simulink model "microgrid_4dg"  (R2025a)
settings: Solver=FixedStepDiscrete  StartTime=0.0  StopTime=0.4  FixedStep=2.5e-06  RelTol=1e-3
libraries: spsThreePhaseSeriesRLCBranchLib x16, spsNeutralLib x10, spsThreePhaseBreakerLib x9, spsThreePhaseVIMeasurementLib x8, spsPWMGenerator2LevelLib x4, spsDCVoltageSourceLib x4, spsUniversalBridgeLib x4, spsGroundLib x1, spspowerguiLib x1
settings Model: Creator=mahmudakon  LastModifiedBy=mahmudakon

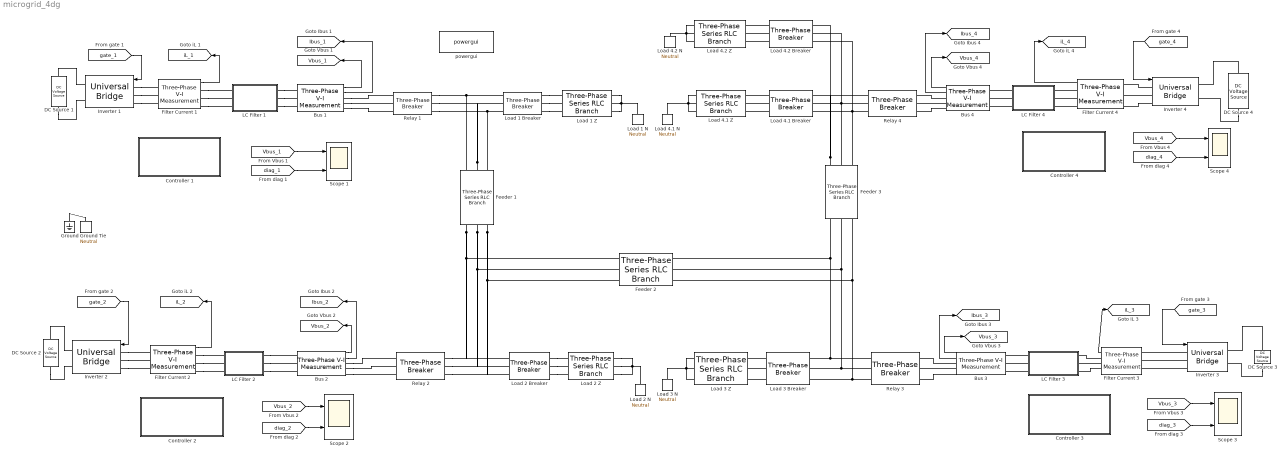
== system microgrid_4dg ==
  Bus {1..4} (4 alike) : spsThreePhaseVIMeasurementLib/Three-Phase V-I Measurement  VoltageMeasurement=phase-to-ground  SetLabelV=off  LabelV=Vabc  Vpu=off  VpuLL=off  CurrentMeasurement=yes  SetLabelI=off  LabelI=Iabc  Ipu=off  Pbase=100e6  Vbase=500e3  OutputType=Complex  PhasorSimulation=off  PSBequivalent=0
  Controller 1 : Subsystem
  Controller 2 : Subsystem
  Controller 3 : Subsystem
  Controller 4 : Subsystem
  DC Source {1..4} (4 alike) : spsDCVoltageSourceLib/DC Voltage Source  Amplitude=45  Measurements=None
  Feeder 1 : spsThreePhaseSeriesRLCBranchLib/Three-Phase Series RLC Branch  LConnTagsString=A|B|C  RConnTagsString=A|B|C  BranchType=RL  Resistance=0.13  Inductance=3.3e-6  Capacitance=1e-6  Measurements=None
  Feeder 2 : spsThreePhaseSeriesRLCBranchLib/Three-Phase Series RLC Branch  LConnTagsString=A|B|C  RConnTagsString=A|B|C  BranchType=RL  Resistance=0.13  Inductance=3.3e-6  Capacitance=1e-6  Measurements=None
  Feeder 3 : spsThreePhaseSeriesRLCBranchLib/Three-Phase Series RLC Branch  LConnTagsString=A|B|C  RConnTagsString=A|B|C  BranchType=RL  Resistance=0.13  Inductance=3.3e-6  Capacitance=1e-6  Measurements=None
  Filter Current {1..4} (4 alike) : spsThreePhaseVIMeasurementLib/Three-Phase V-I Measurement  VoltageMeasurement=no  SetLabelV=off  LabelV=Vabc  Vpu=off  VpuLL=off  CurrentMeasurement=yes  SetLabelI=off  LabelI=Iabc  Ipu=off  Pbase=100e6  Vbase=500e3  OutputType=Complex  PhasorSimulation=off  PSBequivalent=0
  Ground : spsGroundLib/Ground  LConnTagsString=a
  Ground Tie : spsNeutralLib/Neutral  LConnTagsString=a  NodeNumber=1
      settings: AttributesFormatString=node %<NodeNumber>  LibrarySourceBlock=sps_lib/Utilities/Neutral
  Inverter {1..4} (4 alike) : spsUniversalBridgeLib/Universal Bridge  Arms=3  SnubberResistance=1e5  SnubberCapacitance=inf  Device=IGBT / Diodes  Ron=1e-3  Lon=0  ForwardVoltages="[  0  0  ]"  ForwardVoltage=0  GTOparameters=[ 10e-6 , 20e-6 ]  IGBTparameters=[ 1e-6 , 2e-6 ]  Measurements=None  Measurements_2=None  converterType=Rectifier
  LC Filter 1 : Subsystem
  LC Filter 2 : Subsystem
  LC Filter 3 : Subsystem
  LC Filter 4 : Subsystem
  Load 1 Breaker : spsThreePhaseBreakerLib/Three-Phase Breaker  InitialState=closed  SwitchA=on  SwitchB=on  SwitchC=on  SwitchTimes=[1e6]  External=off  BreakerResistance=0.01  SnubberResistance=1e6  SnubberCapacitance=inf  Measurements=None
  Load 1 N : spsNeutralLib/Neutral  LConnTagsString=a  NodeNumber=1
      settings: AttributesFormatString=node %<NodeNumber>  LibrarySourceBlock=sps_lib/Utilities/Neutral
  Load 1 Z : spsThreePhaseSeriesRLCBranchLib/Three-Phase Series RLC Branch  LConnTagsString=A|B|C  RConnTagsString=A|B|C  BranchType=RL  Resistance=10.08  Inductance=6.25e-3  Capacitance=1e-6  Measurements=None
  Load 2 Breaker : spsThreePhaseBreakerLib/Three-Phase Breaker  InitialState=closed  SwitchA=on  SwitchB=on  SwitchC=on  SwitchTimes=[1e6]  External=off  BreakerResistance=0.01  SnubberResistance=1e6  SnubberCapacitance=inf  Measurements=None
  Load 2 N : spsNeutralLib/Neutral  LConnTagsString=a  NodeNumber=2
      settings: AttributesFormatString=node %<NodeNumber>  LibrarySourceBlock=sps_lib/Utilities/Neutral
  Load 2 Z : spsThreePhaseSeriesRLCBranchLib/Three-Phase Series RLC Branch  LConnTagsString=A|B|C  RConnTagsString=A|B|C  BranchType=RL  Resistance=28.34  Inductance=8.00e-3  Capacitance=1e-6  Measurements=None
  Load 3 Breaker : spsThreePhaseBreakerLib/Three-Phase Breaker  InitialState=closed  SwitchA=on  SwitchB=on  SwitchC=on  SwitchTimes=[1e6]  External=off  BreakerResistance=0.01  SnubberResistance=1e6  SnubberCapacitance=inf  Measurements=None
  Load 3 N : spsNeutralLib/Neutral  LConnTagsString=a  NodeNumber=3
      settings: AttributesFormatString=node %<NodeNumber>  LibrarySourceBlock=sps_lib/Utilities/Neutral
  Load 3 Z : spsThreePhaseSeriesRLCBranchLib/Three-Phase Series RLC Branch  LConnTagsString=A|B|C  RConnTagsString=A|B|C  BranchType=RL  Resistance=25.56  Inductance=1.80e-3  Capacitance=1e-6  Measurements=None
  Load 4.1 Breaker : spsThreePhaseBreakerLib/Three-Phase Breaker  InitialState=closed  SwitchA=on  SwitchB=on  SwitchC=on  SwitchTimes=[1e6]  External=off  BreakerResistance=0.01  SnubberResistance=1e6  SnubberCapacitance=inf  Measurements=None
  Load 4.1 N : spsNeutralLib/Neutral  LConnTagsString=a  NodeNumber=4
      settings: AttributesFormatString=node %<NodeNumber>  LibrarySourceBlock=sps_lib/Utilities/Neutral
  Load 4.1 Z : spsThreePhaseSeriesRLCBranchLib/Three-Phase Series RLC Branch  LConnTagsString=A|B|C  RConnTagsString=A|B|C  BranchType=RL  Resistance=10.08  Inductance=6.25e-3  Capacitance=1e-6  Measurements=None
  Load 4.2 Breaker : spsThreePhaseBreakerLib/Three-Phase Breaker  InitialState=open  SwitchA=on  SwitchB=on  SwitchC=on  SwitchTimes=0.2  External=off  BreakerResistance=0.01  SnubberResistance=1e6  SnubberCapacitance=inf  Measurements=None
  Load 4.2 N : spsNeutralLib/Neutral  LConnTagsString=a  NodeNumber=4
      settings: AttributesFormatString=node %<NodeNumber>  LibrarySourceBlock=sps_lib/Utilities/Neutral
  Load 4.2 Z : spsThreePhaseSeriesRLCBranchLib/Three-Phase Series RLC Branch  LConnTagsString=A|B|C  RConnTagsString=A|B|C  BranchType=R  Resistance=10  Inductance=1e-3  Capacitance=1e-6  Measurements=None
  Relay {1..4} (4 alike) : spsThreePhaseBreakerLib/Three-Phase Breaker  InitialState=closed  SwitchA=on  SwitchB=on  SwitchC=on  SwitchTimes=[1e6]  External=off  BreakerResistance=0.01  SnubberResistance=1e6  SnubberCapacitance=inf  Measurements=None
  Scope {1..4} (4 alike) : Scope  NumInputPorts=2
      Scope 1 settings: ActiveDisplayYMinimum=12.426421052352524  ActiveDisplayYMaximum=163.05760904851627
      Scope 4 settings: ActiveDisplayYMinimum=-55.5325630889955  ActiveDisplayYMaximum=59.486517619510956
  powergui : spspowerguiLib/powergui  Priority=1  SimulationMode=Discrete  SampleTime=2.5e-06  frequency=60  Iterations=50  frequencyindice=0  Pbase=100e6  ErrMax=1e-4  UnitsV=kV  UnitsW=MW  buscounter=0  FunctionMessages=off  echomessages=off  EnableUseOfTLC=off  CurrentSourceSwitches=off  DisableSnubberDevices=off  DisableRonSwitches=off  DisableVfSwitches=off  DisplayEquations=off  AutomaticDiscreteSolvers=off  SolverType=Tustin/Backward Euler (TBE)  Interpol=off  ExternalGateDelay=off  methode=off  Ts=100  x0status=blocks  SPID=on  SwTol=0  HookPort=off  NonlinearTolerance=1e-4  nMaxIteration=100  ContinueOnMaxIteration=off  RestoreLinks=warning  ResistiveCurrentMeasurement=off  Frange=[0:2:500]  Ylog=off  Xlog=on  ShowGrid=off  save=off  variable=ZData  structure=0  ZoomFFT=off  StartTime=0.0  cycles=1  DisplayStyle=1  fundamental=60  FreqAxis=off  MaxFrequency=1000  frequencyindicesteady=1  RmsSteady=1  display=off
  tag scope: Ibus_1=global, Ibus_2=global, Ibus_3=global, Ibus_4=global, Vbus_1=global, Vbus_2=global, Vbus_3=global, Vbus_4=global, iL_1=global, iL_2=global, iL_3=global, iL_4=global
  wires:
  Filter Current 1/1 -> [iL_1]
  Bus 1/1 -> [Vbus_1]
  Bus 1/2 -> [Ibus_1]
  [gate_1] -> Inverter 1/1
  Filter Current 2/1 -> [iL_2]
  Bus 2/1 -> [Vbus_2]
  Bus 2/2 -> [Ibus_2]
  [gate_2] -> Inverter 2/1
  Filter Current 3/1 -> [iL_3]
  Bus 3/1 -> [Vbus_3]
  Bus 3/2 -> [Ibus_3]
  [gate_3] -> Inverter 3/1
  Filter Current 4/1 -> [iL_4]
  Bus 4/1 -> [Vbus_4]
  Bus 4/2 -> [Ibus_4]
  [gate_4] -> Inverter 4/1
  [Vbus_1] -> Scope 1/1
  [diag_1] -> Scope 1/2
  [Vbus_2] -> Scope 2/1
  [diag_2] -> Scope 2/2
  [Vbus_3] -> Scope 3/1
  [diag_3] -> Scope 3/2
  [Vbus_4] -> Scope 4/1
  [diag_4] -> Scope 4/2
  connections:
  Ground/LConn1 -- Ground Tie/LConn1
  DC Source 1/RConn1 -- Inverter 1/RConn1
  DC Source 1/LConn1 -- Inverter 1/RConn2
  Inverter 1/LConn1 -- Filter Current 1/LConn1
  Filter Current 1/RConn1 -- LC Filter 1/LConn1
  LC Filter 1/RConn1 -- Bus 1/LConn1
  Bus 1/RConn1 -- Relay 1/LConn1
  Inverter 1/LConn2 -- Filter Current 1/LConn2
  Filter Current 1/RConn2 -- LC Filter 1/LConn2
  LC Filter 1/RConn2 -- Bus 1/LConn2
  Bus 1/RConn2 -- Relay 1/LConn2
  Inverter 1/LConn3 -- Filter Current 1/LConn3
  Filter Current 1/RConn3 -- LC Filter 1/LConn3
  LC Filter 1/RConn3 -- Bus 1/LConn3
  Bus 1/RConn3 -- Relay 1/LConn3
  DC Source 2/RConn1 -- Inverter 2/RConn1
  DC Source 2/LConn1 -- Inverter 2/RConn2
  Inverter 2/LConn1 -- Filter Current 2/LConn1
  Filter Current 2/RConn1 -- LC Filter 2/LConn1
  LC Filter 2/RConn1 -- Bus 2/LConn1
  Bus 2/RConn1 -- Relay 2/LConn1
  Inverter 2/LConn2 -- Filter Current 2/LConn2
  Filter Current 2/RConn2 -- LC Filter 2/LConn2
  LC Filter 2/RConn2 -- Bus 2/LConn2
  Bus 2/RConn2 -- Relay 2/LConn2
  Inverter 2/LConn3 -- Filter Current 2/LConn3
  Filter Current 2/RConn3 -- LC Filter 2/LConn3
  LC Filter 2/RConn3 -- Bus 2/LConn3
  Bus 2/RConn3 -- Relay 2/LConn3
  DC Source 3/RConn1 -- Inverter 3/RConn1
  DC Source 3/LConn1 -- Inverter 3/RConn2
  Inverter 3/LConn1 -- Filter Current 3/LConn1
  Filter Current 3/RConn1 -- LC Filter 3/LConn1
  LC Filter 3/RConn1 -- Bus 3/LConn1
  Bus 3/RConn1 -- Relay 3/LConn1
  Inverter 3/LConn2 -- Filter Current 3/LConn2
  Filter Current 3/RConn2 -- LC Filter 3/LConn2
  LC Filter 3/RConn2 -- Bus 3/LConn2
  Bus 3/RConn2 -- Relay 3/LConn2
  Inverter 3/LConn3 -- Filter Current 3/LConn3
  Filter Current 3/RConn3 -- LC Filter 3/LConn3
  LC Filter 3/RConn3 -- Bus 3/LConn3
  Bus 3/RConn3 -- Relay 3/LConn3
  DC Source 4/RConn1 -- Inverter 4/RConn1
  DC Source 4/LConn1 -- Inverter 4/RConn2
  Inverter 4/LConn1 -- Filter Current 4/LConn1
  Filter Current 4/RConn1 -- LC Filter 4/LConn1
  LC Filter 4/RConn1 -- Bus 4/LConn1
  Bus 4/RConn1 -- Relay 4/LConn1
  Inverter 4/LConn2 -- Filter Current 4/LConn2
  Filter Current 4/RConn2 -- LC Filter 4/LConn2
  LC Filter 4/RConn2 -- Bus 4/LConn2
  Bus 4/RConn2 -- Relay 4/LConn2
  Inverter 4/LConn3 -- Filter Current 4/LConn3
  Filter Current 4/RConn3 -- LC Filter 4/LConn3
  LC Filter 4/RConn3 -- Bus 4/LConn3
  Bus 4/RConn3 -- Relay 4/LConn3
  Relay 1/RConn1 -- Load 1 Breaker/LConn1 -- Feeder 1/LConn1
  Feeder 1/RConn1 -- Load 2 Breaker/LConn1 -- Relay 2/RConn1 -- Feeder 2/LConn1
  Feeder 1/LConn2 -- Relay 1/RConn2 -- Load 1 Breaker/LConn2
  Feeder 1/RConn2 -- Load 2 Breaker/LConn2 -- Relay 2/RConn2 -- Feeder 2/LConn2
  Relay 1/RConn3 -- Feeder 1/LConn3 -- Load 1 Breaker/LConn3
  Feeder 1/RConn3 -- Load 2 Breaker/LConn3 -- Relay 2/RConn3 -- Feeder 2/LConn3
  Relay 3/RConn1 -- Feeder 3/LConn1 -- Feeder 2/RConn1 -- Load 3 Breaker/LConn1
  Relay 3/RConn2 -- Feeder 3/LConn2 -- Feeder 2/RConn2 -- Load 3 Breaker/LConn2
  Relay 3/RConn3 -- Feeder 3/LConn3 -- Feeder 2/RConn3 -- Load 3 Breaker/LConn3
  Feeder 3/RConn1 -- Load 4.2 Breaker/LConn1 -- Relay 4/RConn1 -- Load 4.1 Breaker/LConn1
  Relay 4/RConn2 -- Load 4.2 Breaker/LConn2 -- Feeder 3/RConn2 -- Load 4.1 Breaker/LConn2
  Relay 4/RConn3 -- Load 4.2 Breaker/LConn3 -- Load 4.1 Breaker/LConn3 -- Feeder 3/RConn3
  Load 1 Breaker/RConn1 -- Load 1 Z/LConn1
  Load 1 Z/RConn1 -- Load 1 Z/RConn3 -- Load 1 Z/RConn2 -- Load 1 N/LConn1
  Load 1 Breaker/RConn2 -- Load 1 Z/LConn2
  Load 1 Breaker/RConn3 -- Load 1 Z/LConn3
  Load 2 Breaker/RConn1 -- Load 2 Z/LConn1
  Load 2 Z/RConn1 -- Load 2 Z/RConn3 -- Load 2 N/LConn1 -- Load 2 Z/RConn2
  Load 2 Breaker/RConn2 -- Load 2 Z/LConn2
  Load 2 Breaker/RConn3 -- Load 2 Z/LConn3
  Load 3 Breaker/RConn1 -- Load 3 Z/LConn1
  Load 3 Z/RConn1 -- Load 3 N/LConn1 -- Load 3 Z/RConn3 -- Load 3 Z/RConn2
  Load 3 Breaker/RConn2 -- Load 3 Z/LConn2
  Load 3 Breaker/RConn3 -- Load 3 Z/LConn3
  Load 4.1 Breaker/RConn1 -- Load 4.1 Z/LConn1
  Load 4.1 Z/RConn1 -- Load 4.1 N/LConn1 -- Load 4.1 Z/RConn3 -- Load 4.1 Z/RConn2
  Load 4.1 Breaker/RConn2 -- Load 4.1 Z/LConn2
  Load 4.1 Breaker/RConn3 -- Load 4.1 Z/LConn3
  Load 4.2 Breaker/RConn1 -- Load 4.2 Z/LConn1
  Load 4.2 Z/RConn1 -- Load 4.2 Z/RConn3 -- Load 4.2 N/LConn1 -- Load 4.2 Z/RConn2
  Load 4.2 Breaker/RConn2 -- Load 4.2 Z/LConn2
  Load 4.2 Breaker/RConn3 -- Load 4.2 Z/LConn3

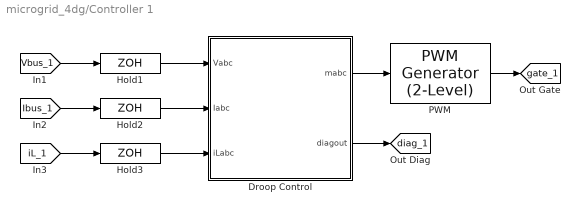
== system microgrid_4dg/Controller 1 ==
  Droop Control : MATLAB Function  TreatAsAtomicUnit=on
  Hold1 : ZeroOrderHold  SampleTime=50e-6
  Hold2 : ZeroOrderHold  SampleTime=50e-6
  Hold3 : ZeroOrderHold  SampleTime=50e-6
  PWM : spsPWMGenerator2LevelLib/PWM Generator (2-Level)  ModulatorType=Three-phase bridge (6 pulses)  ModulatorMode=Unsynchronized  Fc=20000  Pc=90  nF=27  MinMax="[ -1  1 ]"  SamplingTechnique=Natural  ModulatingSignals=off  m=0.8  Freq=60  Phase=0  Ts=0  ShowCarrierOutport=off
  tag scope: diag_1=global, gate_1=global
  wires:
  Hold3/1 -> Droop Control/3(iLabc)
  Droop Control/1(mabc) -> PWM/1
  [iL_1] -> Hold3/1
  Hold1/1 -> Droop Control/1(Vabc)
  [Ibus_1] -> Hold2/1
  Droop Control/2(diagout) -> [diag_1]
  Hold2/1 -> Droop Control/2(Iabc)
  PWM/1 -> [gate_1]
  [Vbus_1] -> Hold1/1

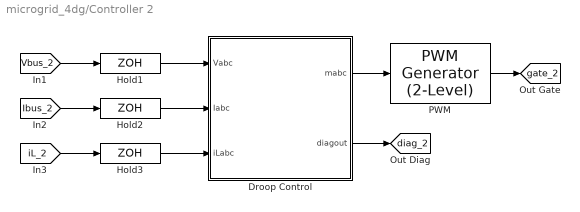
== system microgrid_4dg/Controller 2 ==
  Droop Control : MATLAB Function  TreatAsAtomicUnit=on
  Hold1 : ZeroOrderHold  SampleTime=50e-6
  Hold2 : ZeroOrderHold  SampleTime=50e-6
  Hold3 : ZeroOrderHold  SampleTime=50e-6
  PWM : spsPWMGenerator2LevelLib/PWM Generator (2-Level)  ModulatorType=Three-phase bridge (6 pulses)  ModulatorMode=Unsynchronized  Fc=20000  Pc=90  nF=27  MinMax="[ -1  1 ]"  SamplingTechnique=Natural  ModulatingSignals=off  m=0.8  Freq=60  Phase=0  Ts=0  ShowCarrierOutport=off
  tag scope: diag_2=global, gate_2=global
  wires:
  Hold3/1 -> Droop Control/3(iLabc)
  Droop Control/2(diagout) -> [diag_2]
  [iL_2] -> Hold3/1
  Droop Control/1(mabc) -> PWM/1
  Hold1/1 -> Droop Control/1(Vabc)
  [Ibus_2] -> Hold2/1
  Hold2/1 -> Droop Control/2(Iabc)
  PWM/1 -> [gate_2]
  [Vbus_2] -> Hold1/1

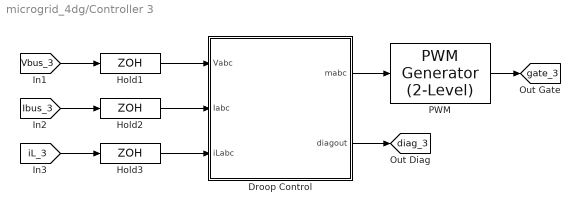
== system microgrid_4dg/Controller 3 ==
  Droop Control : MATLAB Function  TreatAsAtomicUnit=on
  Hold1 : ZeroOrderHold  SampleTime=50e-6
  Hold2 : ZeroOrderHold  SampleTime=50e-6
  Hold3 : ZeroOrderHold  SampleTime=50e-6
  PWM : spsPWMGenerator2LevelLib/PWM Generator (2-Level)  ModulatorType=Three-phase bridge (6 pulses)  ModulatorMode=Unsynchronized  Fc=20000  Pc=90  nF=27  MinMax="[ -1  1 ]"  SamplingTechnique=Natural  ModulatingSignals=off  m=0.8  Freq=60  Phase=0  Ts=0  ShowCarrierOutport=off
  tag scope: diag_3=global, gate_3=global
  wires:
  Hold3/1 -> Droop Control/3(iLabc)
  Droop Control/2(diagout) -> [diag_3]
  [iL_3] -> Hold3/1
  Droop Control/1(mabc) -> PWM/1
  Hold1/1 -> Droop Control/1(Vabc)
  [Ibus_3] -> Hold2/1
  Hold2/1 -> Droop Control/2(Iabc)
  PWM/1 -> [gate_3]
  [Vbus_3] -> Hold1/1

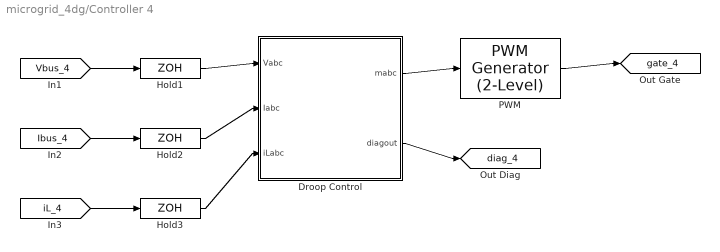
== system microgrid_4dg/Controller 4 ==
  Droop Control : MATLAB Function  TreatAsAtomicUnit=on
  Hold1 : ZeroOrderHold  SampleTime=50e-6
  Hold2 : ZeroOrderHold  SampleTime=50e-6
  Hold3 : ZeroOrderHold  SampleTime=50e-6
  PWM : spsPWMGenerator2LevelLib/PWM Generator (2-Level)  ModulatorType=Three-phase bridge (6 pulses)  ModulatorMode=Unsynchronized  Fc=20000  Pc=90  nF=27  MinMax="[ -1  1 ]"  SamplingTechnique=Natural  ModulatingSignals=off  m=0.8  Freq=60  Phase=0  Ts=0  ShowCarrierOutport=off
  tag scope: diag_4=global, gate_4=global
  wires:
  [Vbus_4] -> Hold1/1
  [Ibus_4] -> Hold2/1
  [iL_4] -> Hold3/1
  Hold1/1 -> Droop Control/1(Vabc)
  Hold2/1 -> Droop Control/2(Iabc)
  Hold3/1 -> Droop Control/3(iLabc)
  Droop Control/1(mabc) -> PWM/1
  PWM/1 -> [gate_4]
  Droop Control/2(diagout) -> [diag_4]

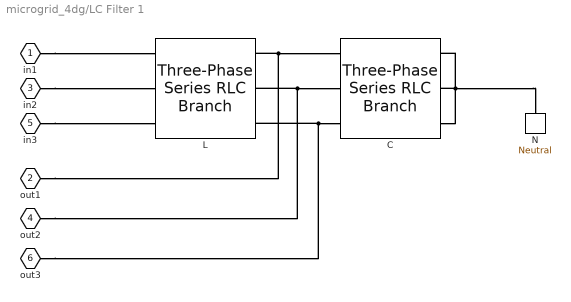
== system microgrid_4dg/LC Filter 1 ==
  C : spsThreePhaseSeriesRLCBranchLib/Three-Phase Series RLC Branch  LConnTagsString=A|B|C  RConnTagsString=A|B|C  BranchType=C  Resistance=1  Inductance=1e-3  Capacitance=22e-6  Measurements=None
  L : spsThreePhaseSeriesRLCBranchLib/Three-Phase Series RLC Branch  LConnTagsString=A|B|C  RConnTagsString=A|B|C  BranchType=L  Resistance=1  Inductance=0.56e-3  Capacitance=1e-6  Measurements=None
  N : spsNeutralLib/Neutral  LConnTagsString=a  NodeNumber=1
      settings: AttributesFormatString=node %<NodeNumber>  LibrarySourceBlock=sps_lib/Utilities/Neutral
  in1 : PMIOPort  Side=Left
  out1 : PMIOPort  Port=2  Side=Right
  in2 : PMIOPort  Port=3  Side=Left
  out2 : PMIOPort  Port=4  Side=Right
  in3 : PMIOPort  Port=5  Side=Left
  out3 : PMIOPort  Port=6  Side=Right
  connections:
  out2/RConn1 -- C/LConn2 -- L/RConn2
  out1/RConn1 -- C/LConn1 -- L/RConn1
  in3/RConn1 -- L/LConn3
  in2/RConn1 -- L/LConn2
  out3/RConn1 -- L/RConn3 -- C/LConn3
  C/RConn3 -- N/LConn1 -- C/RConn1 -- C/RConn2
  in1/RConn1 -- L/LConn1

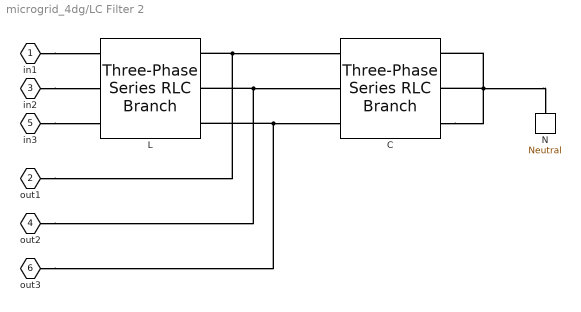
== system microgrid_4dg/LC Filter 2 ==
  C : spsThreePhaseSeriesRLCBranchLib/Three-Phase Series RLC Branch  LConnTagsString=A|B|C  RConnTagsString=A|B|C  BranchType=C  Resistance=1  Inductance=1e-3  Capacitance=22e-6  Measurements=None
  L : spsThreePhaseSeriesRLCBranchLib/Three-Phase Series RLC Branch  LConnTagsString=A|B|C  RConnTagsString=A|B|C  BranchType=L  Resistance=1  Inductance=0.56e-3  Capacitance=1e-6  Measurements=None
  N : spsNeutralLib/Neutral  LConnTagsString=a  NodeNumber=2
      settings: AttributesFormatString=node %<NodeNumber>  LibrarySourceBlock=sps_lib/Utilities/Neutral
  in1 : PMIOPort  Side=Left
  out1 : PMIOPort  Port=2  Side=Right
  in2 : PMIOPort  Port=3  Side=Left
  out2 : PMIOPort  Port=4  Side=Right
  in3 : PMIOPort  Port=5  Side=Left
  out3 : PMIOPort  Port=6  Side=Right
  connections:
  out3/RConn1 -- C/LConn3 -- L/RConn3
  out2/RConn1 -- C/LConn2 -- L/RConn2
  out1/RConn1 -- L/RConn1 -- C/LConn1
  in3/RConn1 -- L/LConn3
  in2/RConn1 -- L/LConn2
  C/RConn3 -- N/LConn1 -- C/RConn1 -- C/RConn2
  in1/RConn1 -- L/LConn1

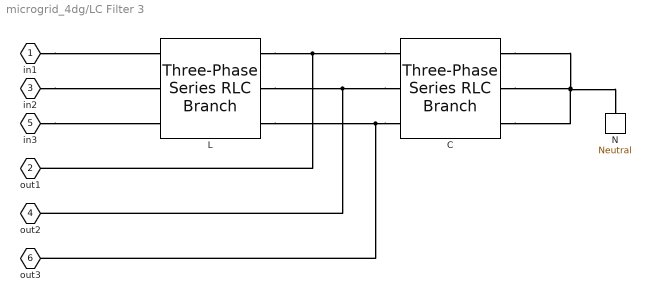
== system microgrid_4dg/LC Filter 3 ==
  C : spsThreePhaseSeriesRLCBranchLib/Three-Phase Series RLC Branch  LConnTagsString=A|B|C  RConnTagsString=A|B|C  BranchType=C  Resistance=1  Inductance=1e-3  Capacitance=22e-6  Measurements=None
  L : spsThreePhaseSeriesRLCBranchLib/Three-Phase Series RLC Branch  LConnTagsString=A|B|C  RConnTagsString=A|B|C  BranchType=L  Resistance=1  Inductance=0.56e-3  Capacitance=1e-6  Measurements=None
  N : spsNeutralLib/Neutral  LConnTagsString=a  NodeNumber=3
      settings: AttributesFormatString=node %<NodeNumber>  LibrarySourceBlock=sps_lib/Utilities/Neutral
  in1 : PMIOPort  Side=Left
  out1 : PMIOPort  Port=2  Side=Right
  in2 : PMIOPort  Port=3  Side=Left
  out2 : PMIOPort  Port=4  Side=Right
  in3 : PMIOPort  Port=5  Side=Left
  out3 : PMIOPort  Port=6  Side=Right
  connections:
  in1/RConn1 -- L/LConn1
  C/LConn1 -- L/RConn1 -- out1/RConn1
  C/RConn1 -- C/RConn3 -- N/LConn1 -- C/RConn2
  in2/RConn1 -- L/LConn2
  C/LConn2 -- L/RConn2 -- out2/RConn1
  in3/RConn1 -- L/LConn3
  C/LConn3 -- L/RConn3 -- out3/RConn1

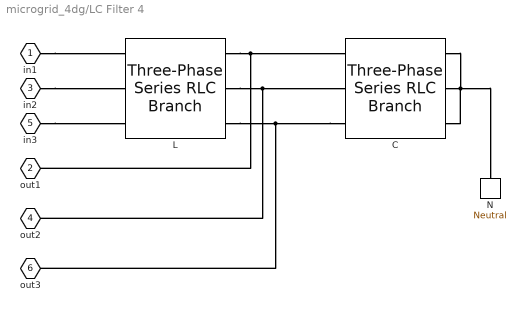
== system microgrid_4dg/LC Filter 4 ==
  C : spsThreePhaseSeriesRLCBranchLib/Three-Phase Series RLC Branch  LConnTagsString=A|B|C  RConnTagsString=A|B|C  BranchType=C  Resistance=1  Inductance=1e-3  Capacitance=22e-6  Measurements=None
  L : spsThreePhaseSeriesRLCBranchLib/Three-Phase Series RLC Branch  LConnTagsString=A|B|C  RConnTagsString=A|B|C  BranchType=L  Resistance=1  Inductance=0.56e-3  Capacitance=1e-6  Measurements=None
  N : spsNeutralLib/Neutral  LConnTagsString=a  NodeNumber=4
      settings: AttributesFormatString=node %<NodeNumber>  LibrarySourceBlock=sps_lib/Utilities/Neutral
  in1 : PMIOPort  Side=Left
  out1 : PMIOPort  Port=2  Side=Right
  in2 : PMIOPort  Port=3  Side=Left
  out2 : PMIOPort  Port=4  Side=Right
  in3 : PMIOPort  Port=5  Side=Left
  out3 : PMIOPort  Port=6  Side=Right
  connections:
  in1/RConn1 -- L/LConn1
  L/RConn1 -- C/LConn1 -- out1/RConn1
  C/RConn1 -- N/LConn1 -- C/RConn3 -- C/RConn2
  in2/RConn1 -- L/LConn2
  L/RConn2 -- C/LConn2 -- out2/RConn1
  in3/RConn1 -- L/LConn3
  C/LConn3 -- out3/RConn1 -- L/RConn3

== matlab function microgrid_4dg/Controller 2/Droop Control ==
  data: Vabc input; mabc output; Iabc input; iLabc input; diagout output
function [mabc, diagout] = dgctrl(Vabc, Iabc, iLabc)
persistent theta Pf Qf intVd intVq intId intIq inited
if isempty(inited)
    theta = 0; Pf = 0; Qf = 0;
    intVd = 0; intVq = 0; intId = 0; intIq = 0;
    inited = true;
end
dt = 5e-05;
w0 = 2*pi*60;
Vdc = 45;
Vnom = 18;
Lf = 0.00056;
Cf = 2.2e-05;
mp = 0.009424777961;
nq = 0.006;
wc = 2*pi*1;
kpv = 0.5; kiv = 200;
kpi = 15;  kii = 4000;
Lv = 0.003;   % virtual series inductance (Pogaku-style virtual impedance)
Kad = 0.5;  % active-damping gain on capacitor current (LC resonance damping)

[Vd, Vq]   = abc2dq(Vabc, theta);
[Id, Iq]   = abc2dq(Iabc, theta);
[ILd, ILq] = abc2dq(iLabc, theta);

Pinst = 1.5*(Vd*Id + Vq*Iq);
Qinst = 1.5*(Vq*Id - Vd*Iq);
Pf = Pf + dt*wc*(Pinst - Pf);
Qf = Qf + dt*wc*(Qinst - Qf);

w = w0 - mp*Pf;
Vref = Vnom - nq*Qf;
theta = mod(theta + dt*w, 2*pi);

% Virtual impedance (Rv=0, series Lv): drop = jXv*I in dq, Xv = w*Lv.
% Subtracted from the droop voltage reference before the outer loop error,
% making the apparent line impedance seen by the droop law more inductive
% than the real (near-purely-resistive) feeder.
Xv = w*Lv;
Vdropd = -Xv*Iq;
Vdropq =  Xv*Id;

% Filter-capacitor current from KCL at the LC filter node: Ic = IL - Ibus.
% Active damping: feed back a term proportional to Ic into the current
% reference to damp the LC filter's own (otherwise-undamped) resonance.
ICd = ILd - Id;
ICq = ILq - Iq;

errVd = (Vref - Vdropd) - Vd;
errVq = (0 - Vdropq) - Vq;
intVd = intVd + dt*errVd;
intVq = intVq + dt*errVq;
Irefd = kpv*errVd + kiv*intVd - w*Cf*Vq - Kad*ICd;
Irefq = kpv*errVq + kiv*intVq + w*Cf*Vd - Kad*ICq;

errId = Irefd - ILd;
errIq = Irefq - ILq;
intId = intId + dt*errId;
intIq = intIq + dt*errIq;
Vinvd = kpi*errId + kii*intId - w*Lf*ILq + Vd;
Vinvq = kpi*errIq + kii*intIq + w*Lf*ILd + Vq;

md = 2*Vinvd/Vdc;
mq = 2*Vinvq/Vdc;
mmag = hypot(md, mq);
if mmag > 1
    md = md/mmag; mq = mq/mmag;
end

mabc = dq2abc(md, mq, theta);
diagout = [Pf; Qf; w/(2*pi)];
end

function [d, q] = abc2dq(xabc, theta)
a = xabc(1); b = xabc(2); c = xabc(3);
d =  (2/3)*( a*cos(theta) + b*cos(theta-2*pi/3) + c*cos(theta+2*pi/3) );
q = -(2/3)*( a*sin(theta) + b*sin(theta-2*pi/3) + c*sin(theta+2*pi/3) );
end

function xabc = dq2abc(d, q, theta)
a = d*cos(theta) - q*sin(theta);
b = d*cos(theta-2*pi/3) - q*sin(theta-2*pi/3);
c = d*cos(theta+2*pi/3) - q*sin(theta+2*pi/3);
xabc = [a; b; c];
end

== matlab function microgrid_4dg/Controller 1/Droop Control ==
  data: Vabc input; mabc output; Iabc input; iLabc input; diagout output
function [mabc, diagout] = dgctrl(Vabc, Iabc, iLabc)
persistent theta Pf Qf intVd intVq intId intIq inited
if isempty(inited)
    theta = 0; Pf = 0; Qf = 0;
    intVd = 0; intVq = 0; intId = 0; intIq = 0;
    inited = true;
end
dt = 5e-05;
w0 = 2*pi*60;
Vdc = 45;
Vnom = 18;
Lf = 0.00056;
Cf = 2.2e-05;
mp = 0.009424777961;
nq = 0.006;
wc = 2*pi*1;
kpv = 0.5; kiv = 200;
kpi = 15;  kii = 4000;
Lv = 0.003;   % virtual series inductance (Pogaku-style virtual impedance)
Kad = 0.5;  % active-damping gain on capacitor current (LC resonance damping)

[Vd, Vq]   = abc2dq(Vabc, theta);
[Id, Iq]   = abc2dq(Iabc, theta);
[ILd, ILq] = abc2dq(iLabc, theta);

Pinst = 1.5*(Vd*Id + Vq*Iq);
Qinst = 1.5*(Vq*Id - Vd*Iq);
Pf = Pf + dt*wc*(Pinst - Pf);
Qf = Qf + dt*wc*(Qinst - Qf);

w = w0 - mp*Pf;
Vref = Vnom - nq*Qf;
theta = mod(theta + dt*w, 2*pi);

% Virtual impedance (Rv=0, series Lv): drop = jXv*I in dq, Xv = w*Lv.
% Subtracted from the droop voltage reference before the outer loop error,
% making the apparent line impedance seen by the droop law more inductive
% than the real (near-purely-resistive) feeder.
Xv = w*Lv;
Vdropd = -Xv*Iq;
Vdropq =  Xv*Id;

% Filter-capacitor current from KCL at the LC filter node: Ic = IL - Ibus.
% Active damping: feed back a term proportional to Ic into the current
% reference to damp the LC filter's own (otherwise-undamped) resonance.
ICd = ILd - Id;
ICq = ILq - Iq;

errVd = (Vref - Vdropd) - Vd;
errVq = (0 - Vdropq) - Vq;
intVd = intVd + dt*errVd;
intVq = intVq + dt*errVq;
Irefd = kpv*errVd + kiv*intVd - w*Cf*Vq - Kad*ICd;
Irefq = kpv*errVq + kiv*intVq + w*Cf*Vd - Kad*ICq;

errId = Irefd - ILd;
errIq = Irefq - ILq;
intId = intId + dt*errId;
intIq = intIq + dt*errIq;
Vinvd = kpi*errId + kii*intId - w*Lf*ILq + Vd;
Vinvq = kpi*errIq + kii*intIq + w*Lf*ILd + Vq;

md = 2*Vinvd/Vdc;
mq = 2*Vinvq/Vdc;
mmag = hypot(md, mq);
if mmag > 1
    md = md/mmag; mq = mq/mmag;
end

mabc = dq2abc(md, mq, theta);
diagout = [Pf; Qf; w/(2*pi)];
end

function [d, q] = abc2dq(xabc, theta)
a = xabc(1); b = xabc(2); c = xabc(3);
d =  (2/3)*( a*cos(theta) + b*cos(theta-2*pi/3) + c*cos(theta+2*pi/3) );
q = -(2/3)*( a*sin(theta) + b*sin(theta-2*pi/3) + c*sin(theta+2*pi/3) );
end

function xabc = dq2abc(d, q, theta)
a = d*cos(theta) - q*sin(theta);
b = d*cos(theta-2*pi/3) - q*sin(theta-2*pi/3);
c = d*cos(theta+2*pi/3) - q*sin(theta+2*pi/3);
xabc = [a; b; c];
end

== matlab function microgrid_4dg/Controller 3/Droop Control ==
  data: Vabc input; mabc output; Iabc input; iLabc input; diagout output
function [mabc, diagout] = dgctrl(Vabc, Iabc, iLabc)
persistent theta Pf Qf intVd intVq intId intIq inited
if isempty(inited)
    theta = 0; Pf = 0; Qf = 0;
    intVd = 0; intVq = 0; intId = 0; intIq = 0;
    inited = true;
end
dt = 5e-05;
w0 = 2*pi*60;
Vdc = 45;
Vnom = 18;
Lf = 0.00056;
Cf = 2.2e-05;
mp = 0.009424777961;
nq = 0.006;
wc = 2*pi*1;
kpv = 0.5; kiv = 200;
kpi = 15;  kii = 4000;
Lv = 0.003;   % virtual series inductance (Pogaku-style virtual impedance)
Kad = 0.5;  % active-damping gain on capacitor current (LC resonance damping)

[Vd, Vq]   = abc2dq(Vabc, theta);
[Id, Iq]   = abc2dq(Iabc, theta);
[ILd, ILq] = abc2dq(iLabc, theta);

Pinst = 1.5*(Vd*Id + Vq*Iq);
Qinst = 1.5*(Vq*Id - Vd*Iq);
Pf = Pf + dt*wc*(Pinst - Pf);
Qf = Qf + dt*wc*(Qinst - Qf);

w = w0 - mp*Pf;
Vref = Vnom - nq*Qf;
theta = mod(theta + dt*w, 2*pi);

% Virtual impedance (Rv=0, series Lv): drop = jXv*I in dq, Xv = w*Lv.
% Subtracted from the droop voltage reference before the outer loop error,
% making the apparent line impedance seen by the droop law more inductive
% than the real (near-purely-resistive) feeder.
Xv = w*Lv;
Vdropd = -Xv*Iq;
Vdropq =  Xv*Id;

% Filter-capacitor current from KCL at the LC filter node: Ic = IL - Ibus.
% Active damping: feed back a term proportional to Ic into the current
% reference to damp the LC filter's own (otherwise-undamped) resonance.
ICd = ILd - Id;
ICq = ILq - Iq;

errVd = (Vref - Vdropd) - Vd;
errVq = (0 - Vdropq) - Vq;
intVd = intVd + dt*errVd;
intVq = intVq + dt*errVq;
Irefd = kpv*errVd + kiv*intVd - w*Cf*Vq - Kad*ICd;
Irefq = kpv*errVq + kiv*intVq + w*Cf*Vd - Kad*ICq;

errId = Irefd - ILd;
errIq = Irefq - ILq;
intId = intId + dt*errId;
intIq = intIq + dt*errIq;
Vinvd = kpi*errId + kii*intId - w*Lf*ILq + Vd;
Vinvq = kpi*errIq + kii*intIq + w*Lf*ILd + Vq;

md = 2*Vinvd/Vdc;
mq = 2*Vinvq/Vdc;
mmag = hypot(md, mq);
if mmag > 1
    md = md/mmag; mq = mq/mmag;
end

mabc = dq2abc(md, mq, theta);
diagout = [Pf; Qf; w/(2*pi)];
end

function [d, q] = abc2dq(xabc, theta)
a = xabc(1); b = xabc(2); c = xabc(3);
d =  (2/3)*( a*cos(theta) + b*cos(theta-2*pi/3) + c*cos(theta+2*pi/3) );
q = -(2/3)*( a*sin(theta) + b*sin(theta-2*pi/3) + c*sin(theta+2*pi/3) );
end

function xabc = dq2abc(d, q, theta)
a = d*cos(theta) - q*sin(theta);
b = d*cos(theta-2*pi/3) - q*sin(theta-2*pi/3);
c = d*cos(theta+2*pi/3) - q*sin(theta+2*pi/3);
xabc = [a; b; c];
end

== matlab function microgrid_4dg/Controller 4/Droop Control ==
  data: Vabc input; mabc output; Iabc input; iLabc input; diagout output
function [mabc, diagout] = dgctrl(Vabc, Iabc, iLabc)
persistent theta Pf Qf intVd intVq intId intIq inited
if isempty(inited)
    theta = 0; Pf = 0; Qf = 0;
    intVd = 0; intVq = 0; intId = 0; intIq = 0;
    inited = true;
end
dt = 5e-05;
w0 = 2*pi*60;
Vdc = 45;
Vnom = 18;
Lf = 0.00056;
Cf = 2.2e-05;
mp = 0.009424777961;
nq = 0.006;
wc = 2*pi*1;
kpv = 0.5; kiv = 200;
kpi = 15;  kii = 4000;
Lv = 0.003;   % virtual series inductance (Pogaku-style virtual impedance)
Kad = 0.5;  % active-damping gain on capacitor current (LC resonance damping)

[Vd, Vq]   = abc2dq(Vabc, theta);
[Id, Iq]   = abc2dq(Iabc, theta);
[ILd, ILq] = abc2dq(iLabc, theta);

Pinst = 1.5*(Vd*Id + Vq*Iq);
Qinst = 1.5*(Vq*Id - Vd*Iq);
Pf = Pf + dt*wc*(Pinst - Pf);
Qf = Qf + dt*wc*(Qinst - Qf);

w = w0 - mp*Pf;
Vref = Vnom - nq*Qf;
theta = mod(theta + dt*w, 2*pi);

% Virtual impedance (Rv=0, series Lv): drop = jXv*I in dq, Xv = w*Lv.
% Subtracted from the droop voltage reference before the outer loop error,
% making the apparent line impedance seen by the droop law more inductive
% than the real (near-purely-resistive) feeder.
Xv = w*Lv;
Vdropd = -Xv*Iq;
Vdropq =  Xv*Id;

% Filter-capacitor current from KCL at the LC filter node: Ic = IL - Ibus.
% Active damping: feed back a term proportional to Ic into the current
% reference to damp the LC filter's own (otherwise-undamped) resonance.
ICd = ILd - Id;
ICq = ILq - Iq;

errVd = (Vref - Vdropd) - Vd;
errVq = (0 - Vdropq) - Vq;
intVd = intVd + dt*errVd;
intVq = intVq + dt*errVq;
Irefd = kpv*errVd + kiv*intVd - w*Cf*Vq - Kad*ICd;
Irefq = kpv*errVq + kiv*intVq + w*Cf*Vd - Kad*ICq;

errId = Irefd - ILd;
errIq = Irefq - ILq;
intId = intId + dt*errId;
intIq = intIq + dt*errIq;
Vinvd = kpi*errId + kii*intId - w*Lf*ILq + Vd;
Vinvq = kpi*errIq + kii*intIq + w*Lf*ILd + Vq;

md = 2*Vinvd/Vdc;
mq = 2*Vinvq/Vdc;
mmag = hypot(md, mq);
if mmag > 1
    md = md/mmag; mq = mq/mmag;
end

mabc = dq2abc(md, mq, theta);
diagout = [Pf; Qf; w/(2*pi)];
end

function [d, q] = abc2dq(xabc, theta)
a = xabc(1); b = xabc(2); c = xabc(3);
d =  (2/3)*( a*cos(theta) + b*cos(theta-2*pi/3) + c*cos(theta+2*pi/3) );
q = -(2/3)*( a*sin(theta) + b*sin(theta-2*pi/3) + c*sin(theta+2*pi/3) );
end

function xabc = dq2abc(d, q, theta)
a = d*cos(theta) - q*sin(theta);
b = d*cos(theta-2*pi/3) - q*sin(theta-2*pi/3);
c = d*cos(theta+2*pi/3) - q*sin(theta+2*pi/3);
xabc = [a; b; c];
end
